simulink model "motor_model_23b_lec9"  (R2025b)
settings: Solver=VariableStepAuto  StartTime=0.0  StopTime=14.499206785118437  RelTol=1e-3
values from neighbouring files (symbols this model uses):
  adown = -mu*g    (= -1.962)    [ex_12_FF.m]    (also in ex_12_I.m = -3.924)
  aup = mu*g    (= 1.962)    [ex_12_FF.m]    (also in ex_12_I.m = 3.924)
  B = 0.15    [ex_11.m]    (also in ex_12_FF.m = 0.147; ex_12_I.m = 0.147; leonora_fast_mission_FF.m = 0.147; leonora_fast_mission_FF_real.m = 0.147)
  D = 8.57e-7    (= 8.57e-07)    [ex_11.m]    (also in ex_12_FF.m; ex_12_I.m; leonora_fast_mission_FF.m = [D; piece.D(keep,:)]; leonora_fast_mission_FF_real.m = [D; piece.D(keep,:)])
  den_ctrl = [alpha*Tlead 1]    [ex_12_FF.m]    (also in ex_12_I.m)
  discrete_true = 1    [ex_12_FF.m]    (also in ex_12_I.m)
  gear = 9.6    [ex_11.m]    (also in ex_12_FF.m; ex_12_I.m; tuning_tr.m; untitled.m)
  J = 0.94e-6    (= 9.4e-07)    [ex_11.m]    (also in ex_12_FF.m = 9.623e-06; ex_12_I.m = 9.623e-06; leonora_fast_mission_FF.m = makeJoin(G,centre,(lo+hi)/2); leonora_fast_mission_FF_real.m = makeJoin(G,centre,(lo+hi)/2))
  Kb = Kt    (= 0.008863)    [ex_11.m]    (also in ex_12_FF.m; ex_12_I.m; tuning_tr.m; untitled.m)
  Ki = Kp/tau_I    (= 0.25)    [ex_12_FF.m]    (also in ex_12_I.m; tuning_tr.m = 0.2)
  Kp = 0.008    [ex_11.m]    (also in ex_12_FF.m = 0.04; ex_12_I.m = 0.04; tuning_tr.m = 0.08)
  Kp_acc = 25    [ex_12_FF.m]    (also in ex_12_I.m)
  Kph = 2.07    [ex_12_FF.m]    (also in ex_12_I.m = 3.7)
  Kt = 0.008863    [ex_11.m]    (also in ex_12_FF.m; ex_12_I.m; tuning_tr.m; untitled.m)
  L = 3.57e-3    (= 0.00357)    [ex_11.m]    (also in ex_12_FF.m; ex_12_I.m; tuning_tr.m; untitled.m)
  num_ctrl = [Tlead 1]    [ex_12_FF.m]    (also in ex_12_I.m)
  R = 3.57    [ex_11.m]    (also in ex_12_FF.m; ex_12_I.m; tuning_tr.m; untitled.m)
  r2m = wrad/gear    (= 0.003125)    [ex_11.m]    (also in ex_12_FF.m = 0.00352078125; ex_12_I.m = 0.00352078125; tuning_tr.m = 0.00352078125)
  Ts = 0.001    [ex_11.m]    (also in ex_12_FF.m = 0.008; ex_12_I.m = 0.008; tuning_tr.m = 0.0005; untitled.m = p.Ts)
  wrad = 0.03    [ex_11.m]    (also in ex_12_FF.m = 0.0337995; ex_12_I.m = 0.0337995; tuning_tr.m = 0.0337995)
settings Model: Creator=chr  LastModifiedBy=migue

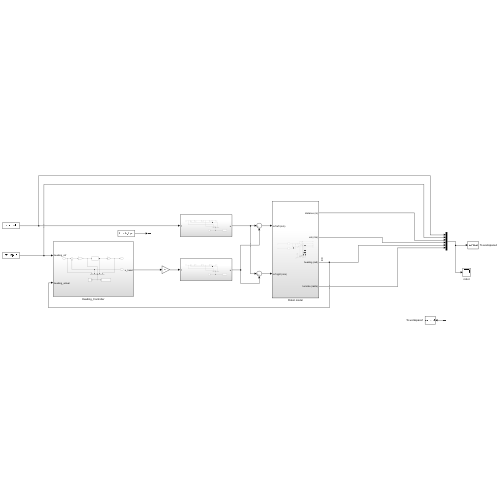
[thumbnail: Simulink's stored preview of the top-level diagram]
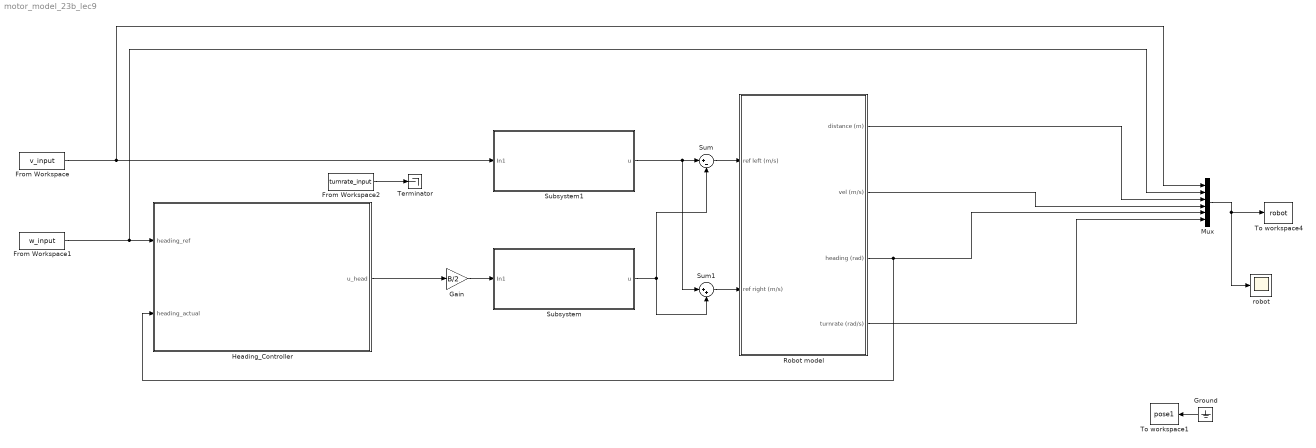
== system motor_model_23b_lec9 ==
  From Workspace : FromWorkspace  VariableName=v_input  Interpolate=off  OutputAfterFinalValue=Holding final value
  From Workspace1 : FromWorkspace  VariableName=w_input  Interpolate=off  OutputAfterFinalValue=Holding final value
  From Workspace2 : FromWorkspace  VariableName=turnrate_input
  Gain : Gain  Gain=B/2
  Ground : Ground
  Heading_Controller : Subsystem
  Mux : Mux  Inputs=6
  Robot model : Subsystem
  Subsystem : Subsystem
  Subsystem1 : Subsystem
  Sum : Sum  Inputs=|+-
  Sum1 : Sum  Inputs=|++
  Terminator : Terminator
  To workspace1 : ToWorkspace  VariableName=pose1  SaveFormat=Timeseries  SampleTime=-1
  To workspace4 : ToWorkspace  VariableName=robot  SaveFormat=Timeseries  SampleTime=-1
  robot : Scope
      settings: ActiveDisplayYMinimum=-1  ActiveDisplayYMaximum=1  DataLoggingVariableName=ScopeData2
  wires:
  Mux/1 -> robot/1, To workspace4/1
  Robot model/4(turnrate (rad/s)) -> Mux/6
  Robot model/3(heading (rad)) -> Heading_Controller/2(heading_actual), Mux/5
  Robot model/2(vel (m/s)) -> Mux/4
  Robot model/1(distance (m)) -> Mux/3
  Sum/1 -> Robot model/1(ref left (m/s))
  From Workspace/1 -> Subsystem1/1(In1), Mux/1
  Sum1/1 -> Robot model/2(ref right (m/s))
  From Workspace1/1 -> Heading_Controller/1(heading_ref), Mux/2
  Gain/1 -> Subsystem/1(In1)
  Subsystem/1(u) -> Sum1/2, Sum/2
  Subsystem1/1(u) -> Sum/1, Sum1/1
  From Workspace2/1 -> Terminator/1
  Heading_Controller/1(u_head) -> Gain/1
  Ground/1 -> To workspace1/1

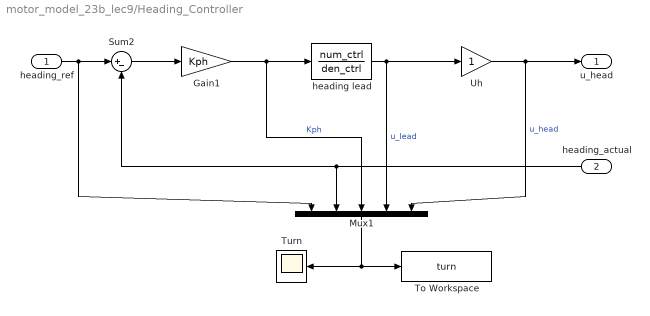
== system motor_model_23b_lec9/Heading_Controller ==
  heading_ref : Inport
  heading_actual : Inport  Port=2
  Gain1 : Gain  Gain=Kph
  Mux1 : Mux  Inputs=5
  Sum2 : Sum  Inputs=|+-
  To Workspace : ToWorkspace  VariableName=turn  SaveFormat=Timeseries  SampleTime=-1
  Turn : Scope
      settings: DataLoggingVariableName=ScopeData3
  Uh : Gain
  heading lead : TransferFcn  Numerator=num_ctrl  Denominator=den_ctrl
  u_head : Outport
  wires:
  Gain1/1 -> heading lead/1, Mux1/3  "Kph"
  Mux1/1 -> Turn/1, To Workspace/1
  heading lead/1 -> Uh/1, Mux1/4  "u_lead"
  heading_ref/1 -> Sum2/1, Mux1/1
  heading_actual/1 -> Mux1/2, Sum2/2
  Sum2/1 -> Gain1/1
  Uh/1 -> Mux1/5, u_head/1  "u_head"

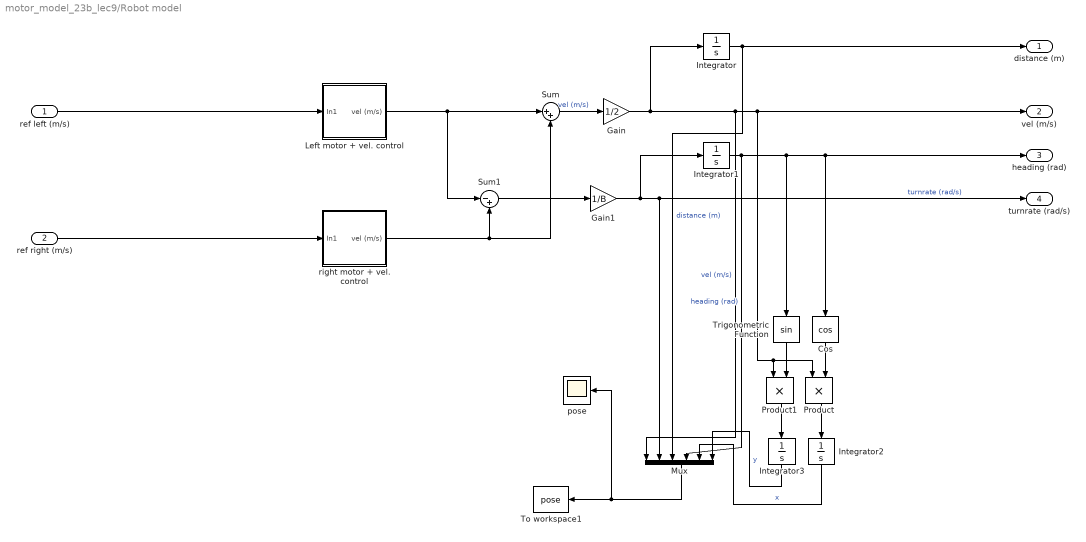
== system motor_model_23b_lec9/Robot model ==
  ref left (m/s) : Inport
  ref right (m/s) : Inport  Port=2
  " right motor + vel. control" : Subsystem
  Cos : Trigonometry  Operator=cos
  Gain : Gain  Gain=1/2
  Gain1 : Gain  Gain=1/B
  Integrator{,1..3} (4 alike) : Integrator
  Left motor + vel. control : Subsystem
  Mux : Mux  Inputs=6
  Product : Product
  Product1 : Product
  Sum : Sum  Inputs=|++
  Sum1 : Sum  Inputs=|-+
  To workspace1 : ToWorkspace  VariableName=pose  SaveFormat=Timeseries  SampleTime=-1
  Trigonometric Function : Trigonometry
  pose : Scope
  distance (m) : Outport
  vel (m/s) : Outport  Port=2
  heading (rad) : Outport  Port=3
  turnrate (rad/s) : Outport  Port=4
  wires:
  Gain1/1 -> Integrator1/1, turnrate (rad/s)/1, Mux/2  "turnrate (rad/s)"
  Sum/1 -> Gain/1  "vel (m/s)"
  Integrator3/1 -> Mux/6  "y"
  " right motor + vel. control"/1(vel (m/s)) -> Sum/2, Sum1/2
  Product/1 -> Integrator2/1
  Mux/1 -> pose/1, To workspace1/1
  Sum1/1 -> Gain1/1
  Integrator2/1 -> Mux/5  "x"
  Cos/1 -> Product/2
  Integrator1/1 -> heading (rad)/1, Cos/1, Trigonometric Function/1, Mux/4  "heading (rad)"
  Left motor + vel. control/1(vel (m/s)) -> Sum1/1, Sum/1
  Product1/1 -> Integrator3/1
  Integrator/1 -> distance (m)/1, Mux/3  "distance (m)"
  Trigonometric Function/1 -> Product1/2
  ref right (m/s)/1 -> " right motor + vel. control"/1(In1)
  ref left (m/s)/1 -> Left motor + vel. control/1(In1)
  Gain/1 -> Mux/1, vel (m/s)/1, Product1/1, Product/1, Integrator/1  "vel (m/s)"

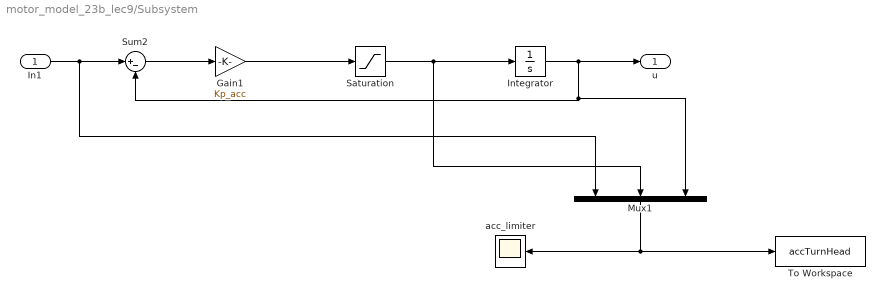
== system motor_model_23b_lec9/Subsystem ==
  In1 : Inport
  Gain1 : Gain  Gain=Kp_acc
  Integrator : Integrator
  Mux1 : Mux  Inputs=3
  Saturation : Saturate  UpperLimit=aup  LowerLimit=adown
  Sum2 : Sum  Inputs=|+-
  To Workspace : ToWorkspace  VariableName=accTurnHead  SaveFormat=Timeseries  SampleTime=-1
  acc_limiter : Scope
      settings: DataLoggingVariableName=ScopeData4
  u : Outport
  wires:
  Integrator/1 -> u/1, Mux1/3, Sum2/2
  In1/1 -> Mux1/1, Sum2/1
  Sum2/1 -> Gain1/1
  Mux1/1 -> acc_limiter/1, To Workspace/1
  Gain1/1 -> Saturation/1
  Saturation/1 -> Integrator/1, Mux1/2

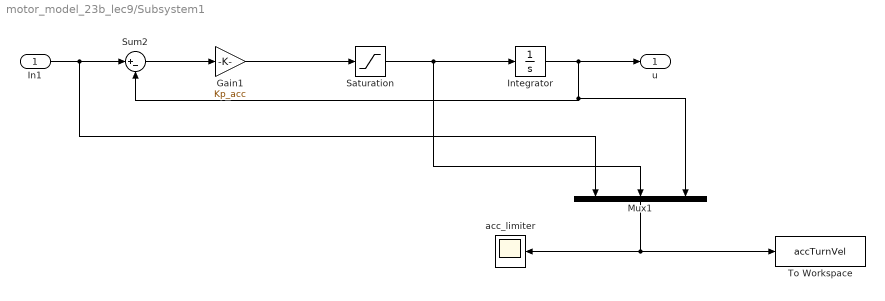
== system motor_model_23b_lec9/Subsystem1 ==
  In1 : Inport
  Gain1 : Gain  Gain=Kp_acc
  Integrator : Integrator
  Mux1 : Mux  Inputs=3
  Saturation : Saturate  UpperLimit=aup  LowerLimit=adown
  Sum2 : Sum  Inputs=|+-
  To Workspace : ToWorkspace  VariableName=accTurnVel  SaveFormat=Timeseries  SampleTime=-1
  acc_limiter : Scope
      settings: DataLoggingVariableName=ScopeData4
  u : Outport
  wires:
  Integrator/1 -> u/1, Mux1/3, Sum2/2
  In1/1 -> Mux1/1, Sum2/1
  Sum2/1 -> Gain1/1
  Mux1/1 -> acc_limiter/1, To Workspace/1
  Gain1/1 -> Saturation/1
  Saturation/1 -> Integrator/1, Mux1/2

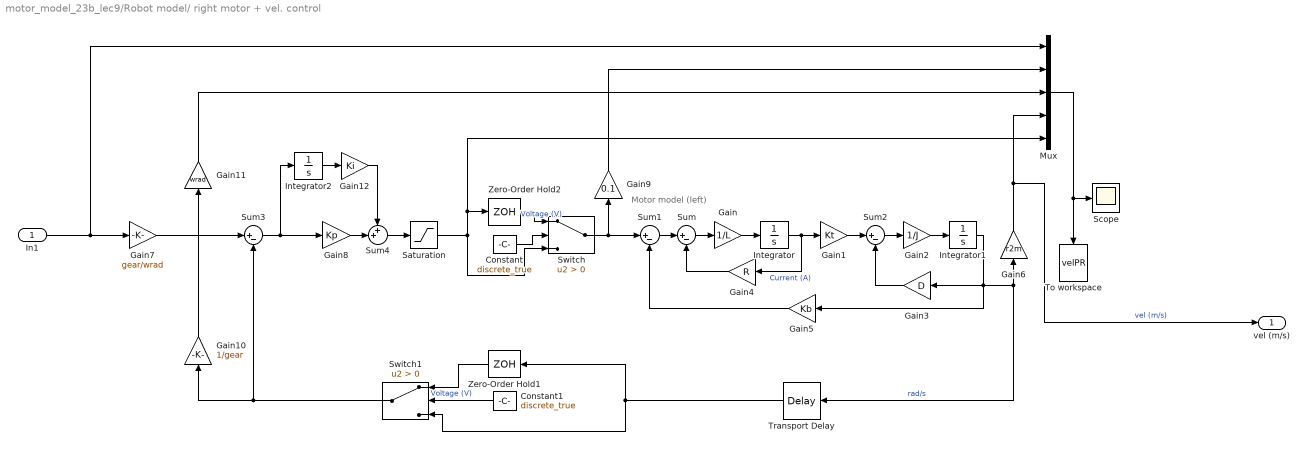
== system motor_model_23b_lec9/Robot model/ right motor + vel. control ==
  note: Motor model (left)
  In1 : Inport
  Constant : Constant  Value=discrete_true
  Constant1 : Constant  Value=discrete_true
  Gain : Gain  Gain=1/L
  Gain1 : Gain  Gain=Kt
  Gain10 : Gain  Gain=1/gear
  Gain11 : Gain  Gain=wrad
  Gain12 : Gain  Gain=Ki
  Gain2 : Gain  Gain=1/J
  Gain3 : Gain  Gain=D
  Gain4 : Gain  Gain=R
  Gain5 : Gain  Gain=Kb
  Gain6 : Gain  Gain=r2m
  Gain7 : Gain  Gain=gear/wrad
  Gain8 : Gain  Gain=Kp
  Gain9 : Gain  Gain=0.1
  Integrator : Integrator
  Integrator1 : Integrator
  Integrator2 : Integrator
  Mux : Mux  Inputs=5
  Saturation : Saturate  UpperLimit=9  LowerLimit=-9
  Scope : Scope
      settings: ActiveDisplayYMinimum=-0.28935  ActiveDisplayYMaximum=6.07084
  Sum{,1..3} (4 alike) : Sum  Inputs=|+-
  Sum4 : Sum  Inputs=++|
  Switch : Switch  Criteria=u2 > Threshold  SaturateOnIntegerOverflow=off  InputSameDT=off
  Switch1 : Switch  Criteria=u2 > Threshold  SaturateOnIntegerOverflow=off  InputSameDT=off
  To workspace : ToWorkspace  VariableName=velPR  SaveFormat=Timeseries  SampleTime=-1
  Transport Delay : TransportDelay  DelayTime=0.01
  Zero-Order Hold1 : ZeroOrderHold  SampleTime=Ts
  Zero-Order Hold2 : ZeroOrderHold  SampleTime=Ts
  vel (m/s) : Outport
  wires:
  Gain6/1 -> vel (m/s)/1, Mux/4  "vel (m/s)"
  Gain3/1 -> Sum2/2
  Integrator/1 -> Gain4/1, Gain1/1  "Current (A)"
  Gain9/1 -> Mux/2
  In1/1 -> Mux/1, Gain7/1
  Integrator1/1 -> Gain3/1, Gain5/1, Transport Delay/1, Gain6/1  "rad/s"
  Gain7/1 -> Sum3/1
  Mux/1 -> Scope/1, To workspace/1
  Sum/1 -> Gain/1
  Saturation/1 -> Switch/3, Mux/5, Zero-Order Hold2/1
  Gain10/1 -> Gain11/1
  Sum1/1 -> Sum/1
  Gain2/1 -> Integrator1/1
  Gain5/1 -> Sum1/2
  Gain1/1 -> Sum2/1
  Sum2/1 -> Gain2/1
  Gain/1 -> Integrator/1
  Gain4/1 -> Sum/2
  Gain11/1 -> Mux/3
  Gain12/1 -> Sum4/1
  Gain8/1 -> Sum4/2
  Integrator2/1 -> Gain12/1
  Sum3/1 -> Gain8/1, Integrator2/1
  Sum4/1 -> Saturation/1
  Constant/1 -> Switch/2
  Zero-Order Hold2/1 -> Switch/1  "Voltage (V)"
  Switch/1 -> Gain9/1, Sum1/1
  Constant1/1 -> Switch1/2
  Zero-Order Hold1/1 -> Switch1/1  "Voltage (V)"
  Transport Delay/1 -> Switch1/3, Zero-Order Hold1/1
  Switch1/1 -> Sum3/2, Gain10/1

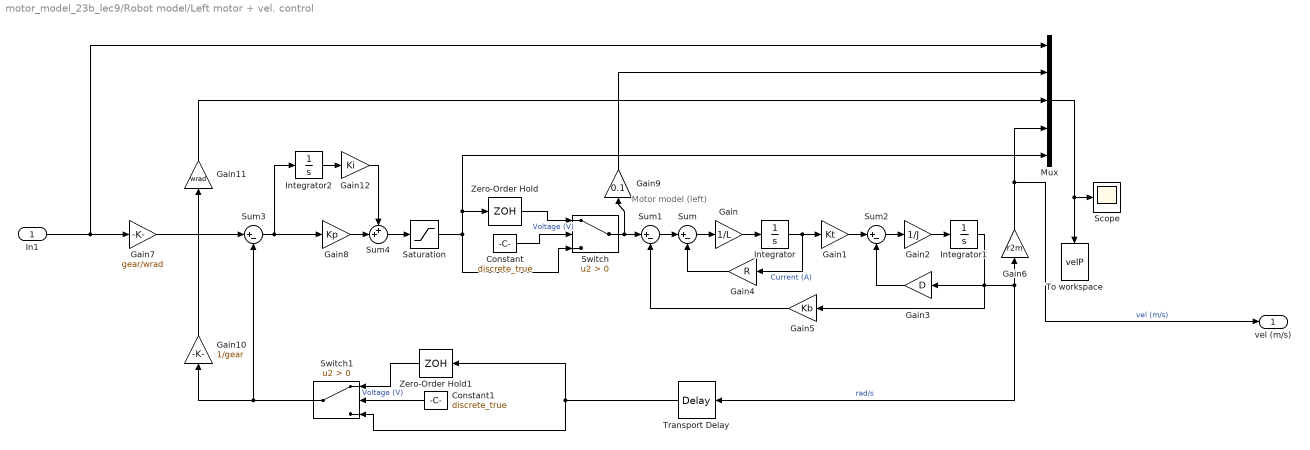
== system motor_model_23b_lec9/Robot model/Left motor + vel. control ==
  note: Motor model (left)
  In1 : Inport
  Constant : Constant  Value=discrete_true
  Constant1 : Constant  Value=discrete_true
  Gain : Gain  Gain=1/L
  Gain1 : Gain  Gain=Kt
  Gain10 : Gain  Gain=1/gear
  Gain11 : Gain  Gain=wrad
  Gain12 : Gain  Gain=Ki
  Gain2 : Gain  Gain=1/J
  Gain3 : Gain  Gain=D
  Gain4 : Gain  Gain=R
  Gain5 : Gain  Gain=Kb
  Gain6 : Gain  Gain=r2m
  Gain7 : Gain  Gain=gear/wrad
  Gain8 : Gain  Gain=Kp
  Gain9 : Gain  Gain=0.1
  Integrator : Integrator
  Integrator1 : Integrator
  Integrator2 : Integrator
  Mux : Mux  Inputs=5
  Saturation : Saturate  UpperLimit=9  LowerLimit=-9
  Scope : Scope
      settings: ActiveDisplayYMinimum=-0.28935  ActiveDisplayYMaximum=6.07084
  Sum{,1..3} (4 alike) : Sum  Inputs=|+-
  Sum4 : Sum  Inputs=++|
  Switch : Switch  Criteria=u2 > Threshold  SaturateOnIntegerOverflow=off  InputSameDT=off
  Switch1 : Switch  Criteria=u2 > Threshold  SaturateOnIntegerOverflow=off  InputSameDT=off
  To workspace : ToWorkspace  VariableName=velP  SaveFormat=Timeseries  SampleTime=-1
  Transport Delay : TransportDelay  DelayTime=0.01
  Zero-Order Hold : ZeroOrderHold  SampleTime=Ts
  Zero-Order Hold1 : ZeroOrderHold  SampleTime=Ts
  vel (m/s) : Outport
  wires:
  Gain6/1 -> vel (m/s)/1, Mux/4  "vel (m/s)"
  Gain3/1 -> Sum2/2
  Integrator/1 -> Gain4/1, Gain1/1  "Current (A)"
  Gain9/1 -> Mux/2
  In1/1 -> Mux/1, Gain7/1
  Integrator1/1 -> Gain3/1, Gain5/1, Transport Delay/1, Gain6/1  "rad/s"
  Sum3/1 -> Integrator2/1, Gain8/1
  Gain7/1 -> Sum3/1
  Mux/1 -> Scope/1, To workspace/1
  Sum/1 -> Gain/1
  Saturation/1 -> Switch/3, Zero-Order Hold/1, Mux/5
  Gain10/1 -> Gain11/1
  Sum1/1 -> Sum/1
  Gain2/1 -> Integrator1/1
  Gain5/1 -> Sum1/2
  Gain1/1 -> Sum2/1
  Sum2/1 -> Gain2/1
  Gain/1 -> Integrator/1
  Gain4/1 -> Sum/2
  Gain11/1 -> Mux/3
  Sum4/1 -> Saturation/1
  Gain8/1 -> Sum4/2
  Gain12/1 -> Sum4/1
  Integrator2/1 -> Gain12/1
  Switch/1 -> Sum1/1, Gain9/1
  Zero-Order Hold/1 -> Switch/1  "Voltage (V)"
  Constant/1 -> Switch/2
  Switch1/1 -> Sum3/2, Gain10/1
  Zero-Order Hold1/1 -> Switch1/1  "Voltage (V)"
  Constant1/1 -> Switch1/2
  Transport Delay/1 -> Zero-Order Hold1/1, Switch1/3
